simulink model "exo_df"  (R2018a)
settings: Solver=FixedStepDiscrete  StartTime=0.0  StopTime=inf  FixedStep=0.001  RelTol=1e-3  EnableMultiTasking=on
InitFcn:
  | init
values from neighbouring files (symbols this model uses):
  motor_saturation_torque = [10.0, 10.0]    [init.m]
  n = 2    [init.m]
  treadmillSpeed = 1.1    [init.m]
undefined symbols (not defined in the file or in its folder): DiscIntNeverNeededParam, Q8, USB
libraries: hdlsllib x50, quarc_library x16, dspsigops x2
(part 2 of 2)

== system exo_df/MOTOR INTERFACE/CAN message encode/Convert float to 12-bit to float3 ==
  x_int : Inport
  x_max : Inport  Port=2
  x_min : Inport  Port=3
  Bit Shift : hdlsllib/Logic and Bit Operations/Bit Shift  mode=Shift Left Logical  N=12
      settings: SourceProductName=HDL Coder  SourceProductBaseCode=HD
  Data Type Conversion : DataTypeConversion  OutDataTypeStr=uint16
  Divide : Product  Inputs=*/
  Product : Product
  Subtract : Sum  Inputs=+-
  Subtract1 : Sum  Inputs=+-
  Subtract2 : Sum  Inputs=+-
  bit : Constant  OutDataTypeStr=uint32
  one : Constant
  float : Outport  VectorParamsAs1DForOutWhenUnconnected=on
  wires:
  Data Type Conversion/1 -> float/1
  Subtract2/1 -> Product/1
  x_int/1 -> Subtract2/1
  Divide/1 -> Product/2
  Subtract/1 -> Divide/2
  Subtract1/1 -> Divide/1
  x_min/1 -> Subtract/2, Subtract2/2
  one/1 -> Subtract1/2
  Bit Shift/1 -> Subtract1/1
  bit/1 -> Bit Shift/1
  Product/1 -> Data Type Conversion/1
  x_max/1 -> Subtract/1

== system exo_df/MOTOR INTERFACE/CAN message encode/Convert float to 16-bit to float ==
  x_int : Inport
  x_max : Inport  Port=2
  x_min : Inport  Port=3
  Bit Shift : hdlsllib/Logic and Bit Operations/Bit Shift  mode=Shift Left Logical  N=16
      settings: SourceProductName=HDL Coder  SourceProductBaseCode=HD
  Data Type Conversion : DataTypeConversion  OutDataTypeStr=uint16
  Divide : Product  Inputs=*/
  Product : Product
  Subtract : Sum  Inputs=+-
  Subtract1 : Sum  Inputs=+-
  Subtract2 : Sum  Inputs=+-
  bit : Constant  OutDataTypeStr=uint32
  one : Constant
  float : Outport  VectorParamsAs1DForOutWhenUnconnected=on
  wires:
  x_max/1 -> Subtract/1
  Product/1 -> Data Type Conversion/1
  bit/1 -> Bit Shift/1
  Bit Shift/1 -> Subtract1/1
  one/1 -> Subtract1/2
  x_min/1 -> Subtract2/2, Subtract/2
  Subtract1/1 -> Divide/1
  Subtract/1 -> Divide/2
  Divide/1 -> Product/2
  x_int/1 -> Subtract2/1
  Subtract2/1 -> Product/1
  Data Type Conversion/1 -> float/1

== system exo_df/MOTOR INTERFACE/CAN message encode1/Convert float to 12-bit to float ==
  x_int : Inport
  x_max : Inport  Port=2
  x_min : Inport  Port=3
  Bit Shift : hdlsllib/Logic and Bit Operations/Bit Shift  mode=Shift Left Logical  N=12
      settings: SourceProductName=HDL Coder  SourceProductBaseCode=HD
  Data Type Conversion : DataTypeConversion  OutDataTypeStr=uint16
  Divide : Product  Inputs=*/
  Product : Product
  Subtract : Sum  Inputs=+-
  Subtract1 : Sum  Inputs=+-
  Subtract2 : Sum  Inputs=+-
  bit : Constant  OutDataTypeStr=uint32
  one : Constant
  float : Outport  VectorParamsAs1DForOutWhenUnconnected=on
  wires:
  x_max/1 -> Subtract/1
  Product/1 -> Data Type Conversion/1
  bit/1 -> Bit Shift/1
  Bit Shift/1 -> Subtract1/1
  one/1 -> Subtract1/2
  x_min/1 -> Subtract2/2, Subtract/2
  Subtract1/1 -> Divide/1
  Subtract/1 -> Divide/2
  Divide/1 -> Product/2
  x_int/1 -> Subtract2/1
  Subtract2/1 -> Product/1
  Data Type Conversion/1 -> float/1

== system exo_df/MOTOR INTERFACE/CAN message encode1/Convert float to 12-bit to float1 ==
  x_int : Inport
  x_max : Inport  Port=2
  x_min : Inport  Port=3
  Bit Shift : hdlsllib/Logic and Bit Operations/Bit Shift  mode=Shift Left Logical  N=12
      settings: SourceProductName=HDL Coder  SourceProductBaseCode=HD
  Data Type Conversion : DataTypeConversion  OutDataTypeStr=uint16
  Divide : Product  Inputs=*/
  Product : Product
  Subtract : Sum  Inputs=+-
  Subtract1 : Sum  Inputs=+-
  Subtract2 : Sum  Inputs=+-
  bit : Constant  OutDataTypeStr=uint32
  one : Constant
  float : Outport  VectorParamsAs1DForOutWhenUnconnected=on
  wires:
  Data Type Conversion/1 -> float/1
  Subtract2/1 -> Product/1
  x_int/1 -> Subtract2/1
  Divide/1 -> Product/2
  Subtract/1 -> Divide/2
  Subtract1/1 -> Divide/1
  x_min/1 -> Subtract/2, Subtract2/2
  one/1 -> Subtract1/2
  Bit Shift/1 -> Subtract1/1
  bit/1 -> Bit Shift/1
  Product/1 -> Data Type Conversion/1
  x_max/1 -> Subtract/1

== system exo_df/MOTOR INTERFACE/CAN message encode1/Convert float to 12-bit to float2 ==
  x_int : Inport
  x_max : Inport  Port=2
  x_min : Inport  Port=3
  Bit Shift : hdlsllib/Logic and Bit Operations/Bit Shift  mode=Shift Left Logical  N=12
      settings: SourceProductName=HDL Coder  SourceProductBaseCode=HD
  Data Type Conversion : DataTypeConversion  OutDataTypeStr=uint16
  Divide : Product  Inputs=*/
  Product : Product
  Subtract : Sum  Inputs=+-
  Subtract1 : Sum  Inputs=+-
  Subtract2 : Sum  Inputs=+-
  bit : Constant  OutDataTypeStr=uint32
  one : Constant
  float : Outport  VectorParamsAs1DForOutWhenUnconnected=on
  wires:
  Data Type Conversion/1 -> float/1
  Subtract2/1 -> Product/1
  x_int/1 -> Subtract2/1
  Divide/1 -> Product/2
  Subtract/1 -> Divide/2
  Subtract1/1 -> Divide/1
  x_min/1 -> Subtract/2, Subtract2/2
  one/1 -> Subtract1/2
  Bit Shift/1 -> Subtract1/1
  bit/1 -> Bit Shift/1
  Product/1 -> Data Type Conversion/1
  x_max/1 -> Subtract/1

== system exo_df/MOTOR INTERFACE/CAN message encode1/Convert float to 12-bit to float3 ==
  x_int : Inport
  x_max : Inport  Port=2
  x_min : Inport  Port=3
  Bit Shift : hdlsllib/Logic and Bit Operations/Bit Shift  mode=Shift Left Logical  N=12
      settings: SourceProductName=HDL Coder  SourceProductBaseCode=HD
  Data Type Conversion : DataTypeConversion  OutDataTypeStr=uint16
  Divide : Product  Inputs=*/
  Product : Product
  Subtract : Sum  Inputs=+-
  Subtract1 : Sum  Inputs=+-
  Subtract2 : Sum  Inputs=+-
  bit : Constant  OutDataTypeStr=uint32
  one : Constant
  float : Outport  VectorParamsAs1DForOutWhenUnconnected=on
  wires:
  x_max/1 -> Subtract/1
  Product/1 -> Data Type Conversion/1
  bit/1 -> Bit Shift/1
  Bit Shift/1 -> Subtract1/1
  one/1 -> Subtract1/2
  x_min/1 -> Subtract2/2, Subtract/2
  Subtract1/1 -> Divide/1
  Subtract/1 -> Divide/2
  Divide/1 -> Product/2
  x_int/1 -> Subtract2/1
  Subtract2/1 -> Product/1
  Data Type Conversion/1 -> float/1

== system exo_df/MOTOR INTERFACE/CAN message encode1/Convert float to 16-bit to float ==
  x_int : Inport
  x_max : Inport  Port=2
  x_min : Inport  Port=3
  Bit Shift : hdlsllib/Logic and Bit Operations/Bit Shift  mode=Shift Left Logical  N=16
      settings: SourceProductName=HDL Coder  SourceProductBaseCode=HD
  Data Type Conversion : DataTypeConversion  OutDataTypeStr=uint16
  Divide : Product  Inputs=*/
  Product : Product
  Subtract : Sum  Inputs=+-
  Subtract1 : Sum  Inputs=+-
  Subtract2 : Sum  Inputs=+-
  bit : Constant  OutDataTypeStr=uint32
  one : Constant
  float : Outport  VectorParamsAs1DForOutWhenUnconnected=on
  wires:
  Data Type Conversion/1 -> float/1
  Subtract2/1 -> Product/1
  x_int/1 -> Subtract2/1
  Divide/1 -> Product/2
  Subtract/1 -> Divide/2
  Subtract1/1 -> Divide/1
  x_min/1 -> Subtract/2, Subtract2/2
  one/1 -> Subtract1/2
  Bit Shift/1 -> Subtract1/1
  bit/1 -> Bit Shift/1
  Product/1 -> Data Type Conversion/1
  x_max/1 -> Subtract/1

== matlab function exo_df/MOTOR INTERFACE/Motor State Handler/MATLAB Function ==
  data: motorReset input; delayedMotorReset output; delayTime input
function delayedMotorReset = fcn(motorReset,delayTime)
persistent count firstCalib

if isempty(count)
    count = 0;
end
if isempty(firstCalib)
    firstCalib = false;
end
delayedMotorReset = 0;

if motorReset == 2
    firstCalib = true;
end

if firstCalib
    if count <= delayTime
        count = count + 1;
    else 
        delayedMotorReset = 1;
    end
end

== matlab function exo_df/MOTOR INTERFACE/Motor State Handler/motorStateHandler1 ==
  data: calibrate input; sigma input; motorStart output; motorStop output; motorResetPos output
function [motorStart, motorStop, motorResetPos] = motorStateHandler(calibrate, sigma)
    % Define constants for readability
    CMD_INACTIVE = 1;
    CMD_ACTIVE = 2;
    
    persistent firstCalibrate sigmaCounter
    if isempty(firstCalibrate), firstCalibrate = 0; end
    if isempty(sigmaCounter), sigmaCounter = 0; end

    wait = 1;  % Duration to hold transitional commands

    % Default outputs
    motorStart = CMD_INACTIVE;
    motorStop = CMD_INACTIVE;
    motorResetPos = CMD_INACTIVE;

    % Calibration logic takes priority
    if calibrate == 1
        if firstCalibrate < wait
            motorStart = CMD_ACTIVE;
            motorResetPos = CMD_INACTIVE;
            motorStop = CMD_INACTIVE;
            firstCalibrate = firstCalibrate + 1;
        elseif firstCalibrate < 2 * wait
            motorStart = CMD_INACTIVE;
            motorResetPos = CMD_ACTIVE;
            motorStop = CMD_INACTIVE;
            firstCalibrate = firstCalibrate + 1;
        else
            motorStart = CMD_INACTIVE;
            motorResetPos = CMD_INACTIVE;
            motorStop = CMD_INACTIVE;
        end
        return  % Skip sigma logic when calibrating
    end

    % If calibration is turned off, reset counter and stop motors
    if calibrate == 0
        firstCalibrate = 0;
        motorStart = CMD_INACTIVE;
        motorResetPos = CMD_INACTIVE;
        motorStop = CMD_ACTIVE;
        return
    end

    % Sigma logic (runs only if calibrate ~= 1)
    if sigma == 0
        sigmaCounter = 0;
        motorStart = CMD_INACTIVE;
        motorResetPos = CMD_INACTIVE;
        motorStop = CMD_ACTIVE;
    elseif sigma == 1
        if sigmaCounter < wait
            motorStart = CMD_ACTIVE;
            motorResetPos = CMD_INACTIVE;
            motorStop = CMD_INACTIVE;
            sigmaCounter = sigmaCounter + 1;
        else
            motorStart = CMD_INACTIVE;
            motorResetPos = CMD_INACTIVE;
            motorStop = CMD_INACTIVE;
        end
    end
end


% function [motorStart, motorStop, motorResetPos]= motorStateHandler(calibrate,sigma)
% persistent firstCalibrate sigmaCounter
% if isempty(firstCalibrate)
%     firstCalibrate = 0;
% end
% if isempty(sigmaCounter)
%     sigmaCounter = 0;
% end
% wait = 2;%2*length(motorIDs);
% motorStart = 1;
% motorResetPos = 1;
% motorStop = 1;
% 
% 
% if sigma == 0
%     motorStart = 1;
%     motorResetPos = 1;
%     motorStop = 2;
%     sigmaCounter = 0;
% end
% 
% if sigma == 1 && sigmaCounter <= wait
%     motorStart = 2;
%     motorResetPos = 1;
%     motorStop = 1;
%     sigmaCounter = sigmaCounter + 1;
%     if sigmaCounter > wait
%         motorStart = 1;
%         motorResetPos = 1;
%         motorStop = 1;
%     end
% end
% 
% 
% if calibrate == 0
%     motorStart = 1;
%     motorResetPos = 1;
%     motorStop = 2;
%     firstCalibrate = 0;
% end
% 
% if calibrate == 1 && firstCalibrate <= wait
%     motorStart = 2;
%     motorResetPos = 1;
%     motorStop = 1;
%     firstCalibrate = firstCalibrate + 1;
%     if firstCalibrate > wait 
%         motorStart = 1;
%         motorResetPos = 2;
%         motorStop = 1;
%         firstCalibrate = firstCalibrate + 1;
%         if firstCalibrate >= 2*wait
%             motorStart = 1;
%             motorResetPos = 1;
%             motorStop = 1;
%         end
%     end
% end
% 
% 
%

== matlab function exo_df/MOTOR INTERFACE/Motor State Handler/motorStateHandler ==
  data: calibrate input; sigma input; motorStart output; motorStop output; motorResetPos output
function [motorStart, motorStop, motorResetPos] = motorStateHandler(calibrate, sigma)
    % Define constants for readability
    CMD_INACTIVE = 1;
    CMD_ACTIVE = 2;
    
    persistent firstCalibrate sigmaCounter
    if isempty(firstCalibrate), firstCalibrate = 0; end
    if isempty(sigmaCounter), sigmaCounter = 0; end

    wait = 1;  % Duration to hold transitional commands

    % Default outputs
    motorStart = CMD_INACTIVE;
    motorStop = CMD_INACTIVE;
    motorResetPos = CMD_INACTIVE;

    % Calibration logic takes priority
    if calibrate == 1
        if firstCalibrate < wait
            motorStart = CMD_ACTIVE;
            motorResetPos = CMD_INACTIVE;
            motorStop = CMD_INACTIVE;
            firstCalibrate = firstCalibrate + 1;
        elseif firstCalibrate < 2 * wait
            motorStart = CMD_INACTIVE;
            motorResetPos = CMD_ACTIVE;
            motorStop = CMD_INACTIVE;
            firstCalibrate = firstCalibrate + 1;
        else
            motorStart = CMD_INACTIVE;
            motorResetPos = CMD_INACTIVE;
            motorStop = CMD_INACTIVE;
        end
        return  % Skip sigma logic when calibrating
    end

    % If calibration is turned off, reset counter and stop motors
    if calibrate == 0
        firstCalibrate = 0;
        motorStart = CMD_INACTIVE;
        motorResetPos = CMD_INACTIVE;
        motorStop = CMD_ACTIVE;
        return
    end

    % Sigma logic (runs only if calibrate ~= 1)
    if sigma == 0
        sigmaCounter = 0;
        motorStart = CMD_INACTIVE;
        motorResetPos = CMD_INACTIVE;
        motorStop = CMD_ACTIVE;
    elseif sigma == 1
        if sigmaCounter < wait
            motorStart = CMD_ACTIVE;
            motorResetPos = CMD_INACTIVE;
            motorStop = CMD_INACTIVE;
            sigmaCounter = sigmaCounter + 1;
        else
            motorStart = CMD_INACTIVE;
            motorResetPos = CMD_INACTIVE;
            motorStop = CMD_INACTIVE;
        end
    end
end


% function [motorStart, motorStop, motorResetPos]= motorStateHandler(calibrate,sigma)
% persistent firstCalibrate sigmaCounter
% if isempty(firstCalibrate)
%     firstCalibrate = 0;
% end
% if isempty(sigmaCounter)
%     sigmaCounter = 0;
% end
% wait = 2;%2*length(motorIDs);
% motorStart = 1;
% motorResetPos = 1;
% motorStop = 1;
% 
% 
% if sigma == 0
%     motorStart = 1;
%     motorResetPos = 1;
%     motorStop = 2;
%     sigmaCounter = 0;
% end
% 
% if sigma == 1 && sigmaCounter <= wait
%     motorStart = 2;
%     motorResetPos = 1;
%     motorStop = 1;
%     sigmaCounter = sigmaCounter + 1;
%     if sigmaCounter > wait
%         motorStart = 1;
%         motorResetPos = 1;
%         motorStop = 1;
%     end
% end
% 
% 
% if calibrate == 0
%     motorStart = 1;
%     motorResetPos = 1;
%     motorStop = 2;
%     firstCalibrate = 0;
% end
% 
% if calibrate == 1 && firstCalibrate <= wait
%     motorStart = 2;
%     motorResetPos = 1;
%     motorStop = 1;
%     firstCalibrate = firstCalibrate + 1;
%     if firstCalibrate > wait 
%         motorStart = 1;
%         motorResetPos = 2;
%         motorStop = 1;
%         firstCalibrate = firstCalibrate + 1;
%         if firstCalibrate >= 2*wait
%             motorStart = 1;
%             motorResetPos = 1;
%             motorStop = 1;
%         end
%     end
% end
% 
% 
%

== matlab function exo_df/MOTOR INTERFACE/Motor State Handler/MATLAB Function3 ==
  data: motorReset input; delayedMotorReset output; delayTime input
function delayedMotorReset = fcn(motorReset,delayTime)
persistent count firstCalib

if isempty(count)
    count = 0;
end
if isempty(firstCalib)
    firstCalib = false;
end
delayedMotorReset = 0;

if motorReset == 2
    firstCalib = true;
end

if firstCalib
    if count <= delayTime
        count = count + 1;
    else 
        delayedMotorReset = 1;
    end
end

== matlab function exo_df/Low-Pass Filter ==
  data: raw_velocity input; old_filtered_velocity input; filtered_velocity output size=[n,1]; velocity_filter_cutoff parameter
function filtered_velocity = low_pass_filter(...
                    raw_velocity, old_filtered_velocity, velocity_filter_cutoff)
filtered_velocity = velocity_filter_cutoff*old_filtered_velocity ...
                + (1 - velocity_filter_cutoff)*raw_velocity;
end

== matlab function exo_df/Treadmill Controller/MATLAB Function ==
  data: runtime input; alpha input; gains input; cmd output; qd_dot input; q input; q_dot input; qd output; qd_dot output
function [cmd,qd,qd_dot] = treadmill(runtime,alpha,gains,qd_dot,q,q_dot)

if runtime <= 0
    qd_dot = 0;
end
qd = qd_dot * runtime / (60*60); 
% qd in miles
% mph = mile/hr, so qd = qd_dot * sec / (60*60)

e = qd - q;
e_dot = qd_dot - q_dot;
r = e_dot + alpha * e;

k1 = gains(1);
k2 = gains(2);
cmd = k1 * r + k2 * sign(r);

== matlab function exo_df/Stop Simulation ==
  data: time input; stopCondition output; simulation_time parameter
function stopCondition = stopSimulation(time, simulation_time)

stopCondition = 0;

if time > simulation_time
    stopCondition = 1;
end

== matlab function exo_df/Treadmill Controller/MATLAB Function1 ==
  data: tick input; tick_unwrapped output; tick_old input; n_old input; n output
function [tick_unwrapped,n] = angle_unwrapped(tick,tick_old,n_old)
n = n_old;
if abs(tick - tick_old) > 0.01
    n = n+1;
end
tick_unwrapped = tick + n*(2^24)*(1/275209/5280);
